simulink model "W08_RC_SineCompare"  (R2024b)
settings: Solver=ode45  StartTime=0.0  StopTime=t_end  MaxStep=0.001  RelTol=1e-3
PreLoadFcn:
  | % W08_RC_SineCompare 기본 파라미터 (모델을 열 때 자동 실행)
  | % 강의자료 3쪽 : R = 100 Ohm, C = 0.001 F -> tau = 0.1 s
  | defs = { 'A_in',1 ; 'w1',2*pi ; 'w3',6*pi ; 't_end',2 ;
  |          'numG',1 ; 'denG',[0.1 1] };
  | for ii = 1:size(defs,1)
  |     if ~evalin('base', sprintf('exist(''%s'',''var'')', defs{ii,1}))
  |         assignin('base', defs{ii,1}, defs{ii,2});
  |     end
  | end
  | clear defs ii
values from neighbouring files (symbols this model uses):
  A_in = 1    [W08_03_run_simulink.m]    (also in W08_04_slide_examples.m = 2; W08_05_rc_simulink.m)
  denG = [tau_1 1]    [W08_05_rc_simulink.m]
  numG = 1    [W08_05_rc_simulink.m]
  w1 = 2*pi    (= 6.28318530718)    [W08_05_rc_simulink.m]
  w3 = 6*pi    (= 18.8495559215)    [W08_05_rc_simulink.m]
settings Model: Creator=admin  LastModifiedBy=admin

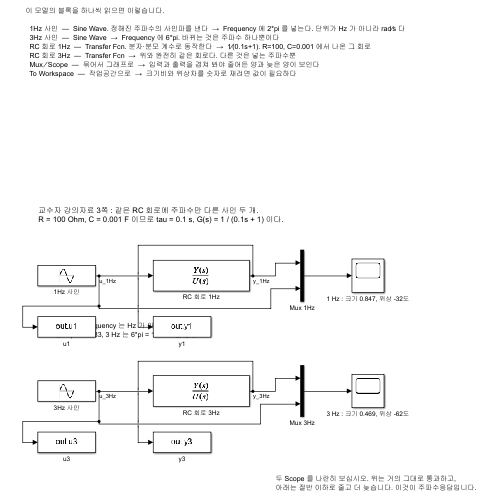
[thumbnail: Simulink's stored preview of the top-level diagram]
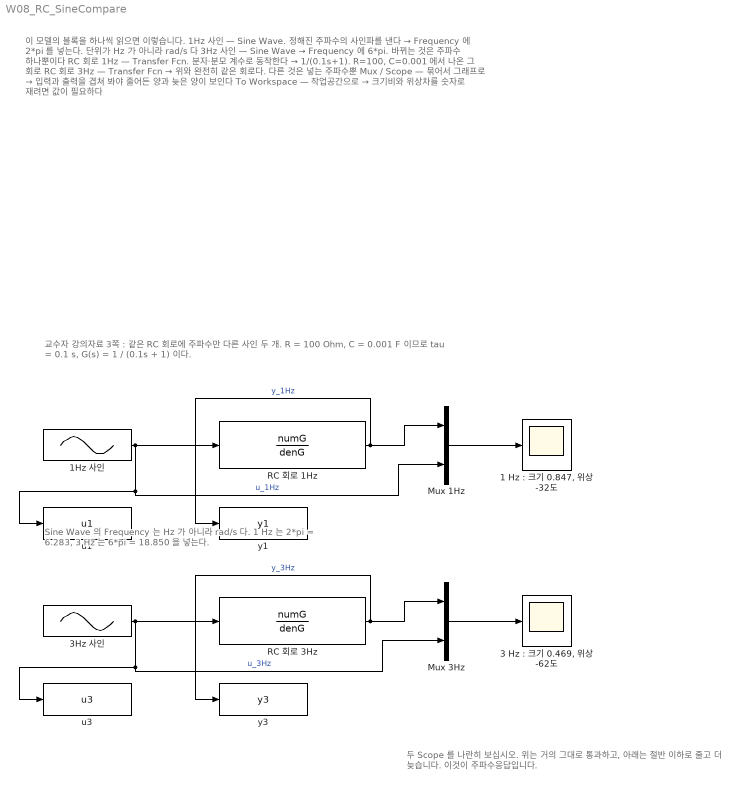
== system W08_RC_SineCompare ==
  note: 교수자 강의자료 3쪽 : 같은 RC 회로에 주파수만 다른 사인 두 개.
      | R = 100 Ohm, C = 0.001 F 이므로 tau = 0.1 s, G(s) = 1 / (0.1s + 1) 이다.
  note: Sine Wave 의 Frequency 는 Hz 가 아니라 rad/s 다.
      | 1 Hz 는 2*pi = 6.283, 3 Hz 는 6*pi = 18.850 을 넣는다.
  note: 두 Scope 를 나란히 보십시오. 위는 거의 그대로 통과하고,
      | 아래는 절반 이하로 줄고 더 늦습니다. 이것이 주파수응답입니다.
  note: 이 모델의 블록을 하나씩 읽으면 이렇습니다.
      |
      |   1Hz 사인  —  Sine Wave. 정해진 주파수의 사인파를 낸다  →  Frequency 에 2*pi 를 넣는다. 단위가 Hz 가 아니라 rad∕s 다
      |   3Hz 사인  —  Sine Wave  →  Frequency 에 6*pi. 바뀌는 것은 주파수 하나뿐이다
      |   RC 회로 1Hz  —  Transfer Fcn. 분자·분모 계수로 동작한다  →  1∕(0.1s+1). R=100, C=0.001 에서 나온 그 회로
      |   RC 회로 3Hz  —  Transfer Fcn  →  위와 완전히 같은 회로다. 다른 것은 넣는 주파수뿐
      |   Mux ∕ Scope  —  묶어서 그래프로  →  입력과 출력을 겹쳐 봐야 줄어든 양과 늦은 양이 보인다
      |   To Workspace  —  작업공간으로  →  크기비와 위상차를 숫자로 재려면 값이 필요하다
  "1 Hz : 크기 0.847, 위상 -32도" : Scope
  1Hz 사인 : Sin  Amplitude=A_in  Frequency=w1  SampleTime=0
  "3 Hz : 크기 0.469, 위상 -62도" : Scope
  3Hz 사인 : Sin  Amplitude=A_in  Frequency=w3  SampleTime=0
  Mux 1Hz : Mux  Inputs=2
  Mux 3Hz : Mux  Inputs=2
  RC 회로 1Hz : TransferFcn  Numerator=numG  Denominator=denG
  RC 회로 3Hz : TransferFcn  Numerator=numG  Denominator=denG
  u1 : ToWorkspace  VariableName=u1  SaveFormat=Timeseries  SampleTime=-1
  u3 : ToWorkspace  VariableName=u3  SaveFormat=Timeseries  SampleTime=-1
  y1 : ToWorkspace  VariableName=y1  SaveFormat=Timeseries  SampleTime=-1
  y3 : ToWorkspace  VariableName=y3  SaveFormat=Timeseries  SampleTime=-1
  wires:
  1Hz 사인/1 -> Mux 1Hz/2, u1/1, RC 회로 1Hz/1  "u_1Hz"
  RC 회로 1Hz/1 -> Mux 1Hz/1, y1/1  "y_1Hz"
  Mux 1Hz/1 -> "1 Hz : 크기 0.847, 위상 -32도"/1
  3Hz 사인/1 -> Mux 3Hz/2, u3/1, RC 회로 3Hz/1  "u_3Hz"
  RC 회로 3Hz/1 -> Mux 3Hz/1, y3/1  "y_3Hz"
  Mux 3Hz/1 -> "3 Hz : 크기 0.469, 위상 -62도"/1
